simulink model "ME598A_Final_Project_R6"  (R2025b)
settings: Solver=ode23t  StartTime=0.0  StopTime=inf  RelTol=1e-3
InitFcn:
  | RPInit
model workspace (MAT data in the model file):
  mapForSim : object (value not decoded)
  occGrid : robotics.BinaryOccupancyGrid (value not decoded)
undefined symbols (not defined in the file): Base, FloorSurface, PlowSurface, Ref, RobotSurface, Side1, Side2, X, Y, Z
libraries: sm_lib x27, nesl_utility x11, RP_Simulator_Components x7, ME598_ProjectLibrary x3, RoboticsPlayground x2
(part 2 of 2)

== stateflow chart ME598A_Final_Project_R6/Chart ==
  state MISSION_MANAGER
    state GO_TO_OBJECT
      entry:
      % Select current object target
      if objects_sorted == 0
      target_x = OBJ1_X;
      target_y = OBJ1_Y;
      else
      target_x = OBJ2_X;
      target_y = OBJ2_Y;
      end
      % Reset color latch for current search
      latched_color = 0;
      last_seen_color = 0;
      stable_color_count = 0;
      during:
      % Compute position and heading to target object
      dx = target_x - xPose;
      dy = target_y - yPose;
      dist = sqrt(dx*dx + dy*dy);
      bearing = atan2(dy, dx);
      heading_error = atan2(sin(bearing - tPose), cos(bearing - tPose));
      % Scale forward speed with distance
      speed = min(28, 10 + 16*dist);
      if speed < 8
      speed = 8;
      end
      % Limit steering correction
      correction = TURN_GAIN * heading_error;
      if correction > 0.65*speed
      correction = 0.65*speed;
      elseif correction < -0.65*speed
      correction = -0.65*speed;
      end
      % Drive toward target object
      left_speed  = speed - correction;
      right_speed = speed + correction;
      % Detect visible unsorted color
      last_seen_color = 0;
      if ~isnan(Red_Distance) && red_sorted == 0
      last_seen_color = 1;
      elseif ~isnan(Green_Distance) && green_sorted == 0
      last_seen_color = 2;
      elseif ~isnan(Blue_Distance) && blue_sorted == 0
      last_seen_color = 3;
      end
      % Count stable detections before latching
      if last_seen_color ~= 0
      stable_color_count = stable_color_count + 1;
      else
      stable_color_count = 0;
      end
    state LATCH_OBJECT
      entry:
      latched_color = last_seen_color;
      if latched_color == 1
      zone_x = RED_ZONE_X;
      zone_y = RED_ZONE_Y;
      elseif latched_color == 2
      zone_x = GREEN_ZONE_X;
      zone_y = GREEN_ZONE_Y;
      elseif latched_color == 3
      zone_x = BLUE_ZONE_X;
      zone_y = BLUE_ZONE_Y;
      else
      zone_x = 0;
      zone_y = 0;
      end
      left_speed = 0;
      right_speed = 0;
      during:
      left_speed = 0;
      right_speed = 0;
    state PUSH_TO_ZONE
      during:
      % Compute vector from robot to target zone
      dx = zone_x - xPose;
      dy = zone_y - yPose;
      dist = sqrt(dx*dx + dy*dy);
      % Compute desired heading toward zone
      bearing = atan2(dy, dx);
      heading_error = atan2(sin(bearing - tPose), cos(bearing - tPose));
      % Use constant forward push speed
      speed = BASE_SPEED;
      % Apply steering correction based on heading error
      correction = DRIVE_GAIN * heading_error;
      % Limit steering so forward motion is maintained
      if correction > 0.6*speed
      correction = 0.6*speed;
      elseif correction < -0.6*speed
      correction = -0.6*speed;
      end
      % Command wheel speeds to push toward zone
      left_speed  = speed - correction;
      right_speed = speed + correction;
    state ALIGN_TO_ZONE
      during:
      % Compute heading from current pose to target zone
      bearing = atan2(zone_y - yPose, zone_x - xPose);
      % Wrap heading error to [-pi, pi]
      heading_error = atan2(sin(bearing - tPose), cos(bearing - tPose));
      % Set turn speed proportional to heading error
      speed = TURN_GAIN * heading_error;
      % Enforce minimum turn speed when not yet aligned
      if abs(speed) < 5 && abs(heading_error) > ALIGN_TOL
      speed = 5 * sign(heading_error);
      end
      % Turn in place toward zone
      left_speed  = -speed;
      right_speed =  speed;
    state INIT
      entry:
      objects_sorted = 0;
      red_sorted = 0;
      green_sorted = 0;
      blue_sorted = 0;
      target_x = OBJ1_X;
      target_y = OBJ1_Y;
      latched_color = 0;
      last_seen_color = 0;
      stable_color_count = 0;
      zone_x = 0;
      zone_y = 0;
      left_speed = 0;
      right_speed = 0;
    state BACK_OUT
      entry:
      % Store starting position for reverse motion
      back_start_x = xPose;
      back_start_y = yPose;
      during:
      % Drive straight backward to clear the object
      left_speed  = -BACK_SPEED;
      right_speed = -BACK_SPEED;
    state MARK_SORTED
      entry:
      % Mark current object as sorted
      if latched_color == 1 && red_sorted == 0
      red_sorted = 1;
      objects_sorted = objects_sorted + 1;
      elseif latched_color == 2 && green_sorted == 0
      green_sorted = 1;
      objects_sorted = objects_sorted + 1;
      elseif latched_color == 3 && blue_sorted == 0
      blue_sorted = 1;
      objects_sorted = objects_sorted + 1;
      end
      % Clear latched detection values
      latched_color = 0;
      last_seen_color = 0;
      stable_color_count = 0;
      % Stop robot in sorted state
      left_speed = 0;
      right_speed = 0;
      during:
      % Hold robot stopped
      left_speed = 0;
      right_speed = 0;
    state STOP
      entry:
      % Stop both wheels on entry
      left_speed = 0;
      right_speed = 0;
      during:
      % Keep robot stopped
      left_speed = 0;
      right_speed = 0;
    state FINAL_ALIGN
      entry:
      % Reset settle counter on entry
      final_settle_count = 0;
      during:
      % Compute heading error relative to final desired angle
      align_error = atan2(sin(0 - tPose), cos(0 - tPose));
      % Command in-place rotation for final alignment
      left_speed  = -FINAL_TURN_GAIN * align_error;
      right_speed =  FINAL_TURN_GAIN * align_error;
      % Count consecutive aligned samples
      if abs(align_error) < FINAL_ALIGN_TOL
      final_settle_count = final_settle_count + 1;
      else
      final_settle_count = 0;
      end
    state RETURN_HOME_DRIVE
      during:
      dx = home_x - xPose;
      dy = home_y - yPose;
      dist = sqrt(dx*dx + dy*dy);
      bearing = atan2(dy, dx);
      heading_error = atan2(sin(bearing - tPose), cos(bearing - tPose));
      speed = min(24, 10 + 18*dist);
      if speed < 6
      speed = 6;
      end
      correction = 14 * heading_error;
      if correction > 0.6*speed
      correction = 0.6*speed;
      elseif correction < -0.6*speed
      correction = -0.6*speed;
      end
      left_speed  = speed - correction;
      right_speed = speed + correction;
    state RETURN_HOME_ALIGN
      during:
      % Compute heading from current pose to home position
      bearing = atan2(home_y - yPose, home_x - xPose);
      % Wrap heading error to [-pi, pi]
      heading_error = atan2(sin(bearing - tPose), cos(bearing - tPose));
      % Set turn speed proportional to heading error
      speed = 20 * heading_error;
      % Enforce minimum turn speed when not yet aligned
      if abs(speed) < 4 && abs(heading_error) > 0.08
      speed = 4 * sign(heading_error);
      end
      % Turn in place toward home
      left_speed  = -speed;
      right_speed =  speed;
    (default) -> INIT
    INIT -> GO_TO_OBJECT : [1]
    GO_TO_OBJECT -> LATCH_OBJECT : [ sqrt((xPose-target_x)^2 + (yPose-target_y)^2) < OBJECT_CAPTURE_RADIUS && stable_color_count >= COLOR_LATCH_COUNT ]
    PUSH_TO_ZONE -> BACK_OUT : [ sqrt((xPose-zone_x)^2 + (yPose-zone_y)^2) < ZONE_REACH_RADIUS ]
    ALIGN_TO_ZONE -> PUSH_TO_ZONE : [abs(atan2(sin(atan2(zone_y - yPose, zone_x - xPose) - tPose), cos(atan2(zone_y - yPose, zone_x - xPose) - tPose))) <= ALIGN_TOL]
    LATCH_OBJECT -> ALIGN_TO_ZONE [order 1] : [latched_color ~= 0]
    BACK_OUT -> MARK_SORTED : [ sqrt((xPose-back_start_x)^2 + (yPose-back_start_y)^2) > BACKOUT_DIST ]
    LATCH_OBJECT -> GO_TO_OBJECT [order 2] : [latched_color == 0]
    MARK_SORTED -> GO_TO_OBJECT [order 1] : [objects_sorted < 2]
    MARK_SORTED -> RETURN_HOME_ALIGN [order 2] : [objects_sorted == 2]
    FINAL_ALIGN -> STOP : [final_settle_count >= FINAL_SETTLE_COUNT]
    RETURN_HOME_DRIVE -> FINAL_ALIGN : [ sqrt((xPose-home_x)^2 + (yPose-home_y)^2) < HOME_RADIUS ]
    RETURN_HOME_ALIGN -> RETURN_HOME_DRIVE : [abs(heading_error) < 0.08]
  state AVOID_WALL
    entry:
    wall_clear_count = 0;
    % Latch escape direction once on entry
    if isnan(Left_Distance)
    left_d = INF_DIST;
    else
    left_d = Left_Distance;
    end
    if isnan(Right_Distance)
    right_d = INF_DIST;
    else
    right_d = Right_Distance;
    end
    % Choose the more open side once
    if left_d > right_d
    escape_dir = 1;     % turn left
    else
    escape_dir = -1;    % turn right
    end
    during:
    if isnan(Front_Distance)
    front_d = INF_DIST;
    else
    front_d = Front_Distance;
    end
    if isnan(Left_Distance)
    left_d = INF_DIST;
    else
    left_d = Left_Distance;
    end
    if isnan(Right_Distance)
    right_d = INF_DIST;
    else
    right_d = Right_Distance;
    end
    % Reactive avoidance with latched direction
    if front_d < WALL_EXIT
    if escape_dir == 1
    left_speed  = -16;
    right_speed =  12;
    else
    left_speed  =  12;
    right_speed = -16;
    end
    elseif left_d < WALL_EXIT
    % left wall close -> turn right
    left_speed  =  14;
    right_speed = -14;
    escape_dir = -1;
    elseif right_d < WALL_EXIT
    % right wall close -> turn left
    left_speed  = -14;
    right_speed =  14;
    escape_dir = 1;
    else
    left_speed  = 0;
    right_speed = 0;
    end
    % Debounced clear condition using sanitized distances
    if (front_d > WALL_EXIT) && (left_d > WALL_EXIT) && (right_d > WALL_EXIT)
    wall_clear_count = wall_clear_count + 1;
    else
    wall_clear_count = 0;
    end
  MISSION_MANAGER -> AVOID_WALL : [ (~isnan(Front_Distance) && Front_Distance < WALL_ENTER) || (~isnan(Left_Distance)  && Left_Distance  < WALL_ENTER) || (~isnan(Right_Distance) && Right_Distance < WALL_ENTER) ]
  (default) -> MISSION_MANAGER
  AVOID_WALL -> (history) : [front_d > WALL_EXIT]
  data: Blue_Distance input; Green_Distance input; Red_Distance input; tPose input; xPose input; yPose input; left_speed output; right_speed output; target_x local =0; target_y local =0; dx local =0; bearing local =0; heading_error local =999; BASE_SPEED local =50; zone_y local =0; zone_x local =0; blue_sorted local =0; green_sorted local =0; red_sorted local =0; objects_sorted local =0; dist local =1; home_x local =0; home_y local =0; align_error local =0; speed local =0; Front_Distance input; Left_Distance input; Right_Distance input; correction local =0; latched_color local =0; last_seen_color local =0; stable_color_count local =0; back_start_x local =0; back_start_y local =0; wall_clear_count local =0; final_settle_count local =0; front_d local =0; left_d local =0; right_d local =0; GREEN_ZONE_Y local =-2.0; BLUE_ZONE_Y local =0.0; RED_ZONE_X local =2.0; RED_ZONE_Y local =2.0; GREEN_ZONE_X local =2.0; TURN_GAIN local =22; BLUE_ZONE_X local =-2.0; ALIGN_TOL local =0.08; BACK_SPEED local =16; DRIVE_GAIN local =14; WALL_EXIT local =0.5; FINAL_ALIGN_TOL local =0.15; FINAL_TURN_GAIN local =18; OBJECT_CAPTURE_RADIUS local =0.2; COLOR_LATCH_COUNT local =3; CLEAR_COUNT_MIN local =5; HOME_RADIUS local =0.18; WALL_ENTER local =0.3; BACKOUT_DIST local =0.55; FINAL_SETTLE_COUNT local =6; ZONE_REACH_RADIUS local =0.45; OBJ1_X local =0; OBJ1_Y local =-1.5; OBJ2_Y local =1.5; OBJ2_X local =0; INF_DIST local =999; dy local =0; MAX_TURN_SPEED local =20; MIN_TURN_SPEED local =0; turn_cmd local; escape_dir local =0

== matlab function ME598A_Final_Project_R6/-180* : 180* ==
  data: deg input; deg output
function deg = degWrap(deg)

% % Convert radians to degrees
% deg = 180/pi * rad;


% Wrap degree value to the range -180* : +180*
for idx = 1:length(deg)
    while deg(idx) < -180
        deg(idx) = deg(idx)+360;
    end
    
    while deg(idx) > 180
        deg(idx) = deg(idx)-360;
    end
end

return
